simulink model "mainPID"  (R2018b)
settings: Solver=ode5  StartTime=0.0  StopTime=10  RelTol=1e-3
InitFcn:
  | init
values from neighbouring files (symbols this model uses):
  AngDisp = [0 1.57079632679 1.57079632679 1.57079632679 1.57079632679 1.57079632679 0]    [MPCerror.mat]    (also in PIDerror.mat; Q_MPC.m = [0,pi/2,pi/2,pi/2,pi/2,pi/2,0]; Q_PID.m = [0,pi/2,pi/2,pi/2,pi/2,pi/2,0])
  AngVel = [0 0 0 0 0 0 0]    [MPCerror.mat]    (also in PIDerror.mat; Q_MPC.m = [0,0,0,0,0,0,0]; Q_PID.m = [0,0,0,0,0,0,0])
  params = [0.2 3 9.149 36.044 9.149 3 0.2 0.1 0.4 0.4 0.625 0.4 ... (31 elements, 1x31)]    [MPCerror.mat]    (also in PIDerror.mat; Q_MPC.m = [m1,m2,m3,m4,m5,m6,m7,L1,L2,L3,L4,L5,L6,L7,L1c,L2c,L3c,L4c,L; Q_PID.m = [m1,m2,m3,m4,m5,m6,m7,L1,L2,L3,L4,L5,L6,L7,L1c,L2c,L3c,L4c,L)
libraries: simulink x1
settings Model: Creator=Negar Pajooh  LastModifiedBy=Negar Pajooh

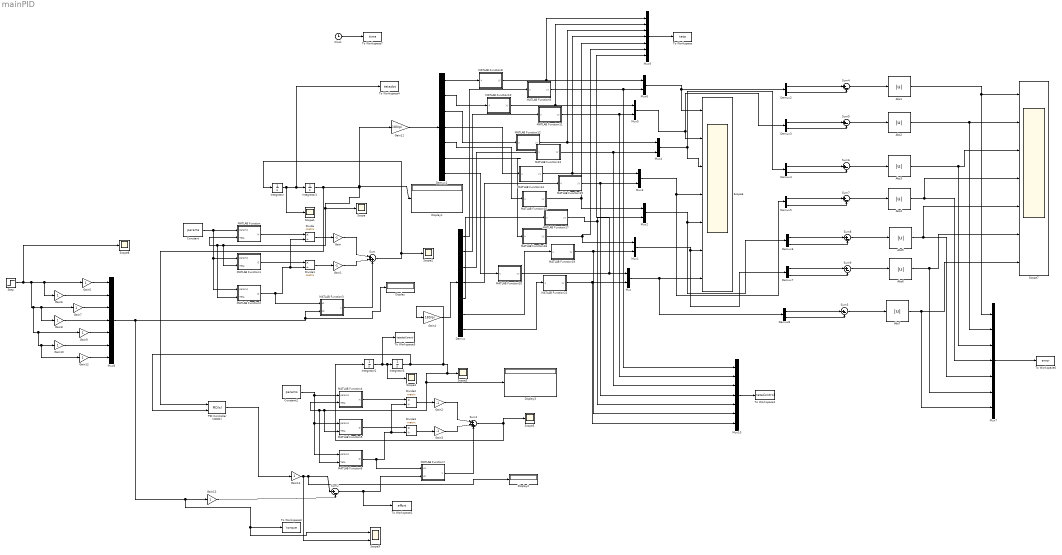
== system mainPID ==
  Abs{1..7} (7 alike) : Abs
  Clock : Clock
  Constant : Constant  Value=params
  Constant2 : Constant  Value=params
  Demux : Demux  Outputs=7
  Demux1 : Demux  Outputs=7
  Demux{2..8} (7 alike) : Demux  Outputs=2
  Display{,1..3} (4 alike) : Display
  Divide{,1..3} (4 alike) : Product  Inputs=*/  Multiplication=Matrix(*)
  Gain{,1..3} (4 alike) : Gain  Gain=-1
  Gain{5..10,12..14} (9 alike) : Gain
  Gain11 : Gain  Gain=180/pi
  Gain4 : Gain  Gain=180/pi
  Integrator : Integrator  InitialCondition=AngVel
  Integrator1 : Integrator  InitialCondition=AngDisp
  Integrator2 : Integrator  InitialCondition=AngVel
  Integrator3 : Integrator  InitialCondition=AngDisp
  MATLAB Function : MATLAB Function  TreatAsAtomicUnit=on
  MATLAB Function1 : MATLAB Function  TreatAsAtomicUnit=on
  MATLAB Function10 : MATLAB Function  TreatAsAtomicUnit=on
  MATLAB Function11 : MATLAB Function  TreatAsAtomicUnit=on
  MATLAB Function12 : MATLAB Function  TreatAsAtomicUnit=on
  MATLAB Function13 : MATLAB Function  TreatAsAtomicUnit=on
  MATLAB Function14 : MATLAB Function  TreatAsAtomicUnit=on
  MATLAB Function15 : MATLAB Function  TreatAsAtomicUnit=on
  MATLAB Function16 : MATLAB Function  TreatAsAtomicUnit=on
  MATLAB Function17 : MATLAB Function  TreatAsAtomicUnit=on
  MATLAB Function18 : MATLAB Function  TreatAsAtomicUnit=on
  MATLAB Function19 : MATLAB Function  TreatAsAtomicUnit=on
  MATLAB Function2 : MATLAB Function  TreatAsAtomicUnit=on
  MATLAB Function20 : MATLAB Function  TreatAsAtomicUnit=on
  MATLAB Function21 : MATLAB Function  TreatAsAtomicUnit=on
  MATLAB Function3 : MATLAB Function  TreatAsAtomicUnit=on
  MATLAB Function4 : MATLAB Function  TreatAsAtomicUnit=on
  MATLAB Function5 : MATLAB Function  TreatAsAtomicUnit=on
  MATLAB Function6 : MATLAB Function  TreatAsAtomicUnit=on
  MATLAB Function7 : MATLAB Function  TreatAsAtomicUnit=on
  MATLAB Function8 : MATLAB Function  TreatAsAtomicUnit=on
  MATLAB Function9 : MATLAB Function  TreatAsAtomicUnit=on
  Mux{,1..6} (7 alike) : Mux  Inputs=2
  Mux{7..10} (4 alike) : Mux  Inputs=7
  PID Controller (2DOF) : simulink/Continuous/PID Controller (2DOF)  Controller=PID  Form=Parallel  TimeDomain=Continuous-time  SampleTime=-1  IntegratorMethod=Forward Euler  FilterMethod=Forward Euler  ControllerParametersSource=internal  P=10  I=0.001  D=0  UseFilter=on  N=100  b=1  c=1  TunerSelectOption=Transfer Function Based (PID Tuner App)  InitialConditionSource=internal  InitialConditionForIntegrator=0  InitialConditionForFilter=0  DifferentiatorICPrevScaledInput=0  ExternalReset=none  TrackingMode=off  Kt=1  LimitOutput=off  UpperSaturationLimit=inf  LowerSaturationLimit=-inf  LinearizeAsGain=on  AntiWindupMode=none  Kb=1  POutMin=[]  POutMax=[]  IOutMin=[]  IOutMax=[]  DOutMin=[]  DOutMax=[]  NOutMin=[]  NOutMax=[]  bOutMin=[]  bOutMax=[]  cOutMin=[]  cOutMax=[]  SumOutMin=[]  SumOutMax=[]  SaturationOutMin=[]  SaturationOutMax=[]  PParamMin=[]  PParamMax=[]  IParamMin=[]  IParamMax=[]  DParamMin=[]  DParamMax=[]  NParamMin=[]  NParamMax=[]  bParamMin=[]  bParamMax=[]  cParamMin=[]  cParamMax=[]  KbParamMin=[]  KbParamMax=[]  KtParamMin=[]  KtParamMax=[]  KbOutMin=[]  KbOutMax=[]  KtOutMin=[]  KtOutMax=[]  IntegratorOutMin=[]  IntegratorOutMax=[]  FilterOutMin=[]  FilterOutMax=[]  SumI1OutMin=[]  SumI1OutMax=[]  SumI2OutMin=[]  SumI2OutMax=[]  SumI3OutMin=[]  SumI3OutMax=[]  SumI4OutMin=[]  SumI4OutMax=[]  SumDOutMin=[]  SumDOutMax=[]  Sum1OutMin=[]  Sum1OutMax=[]  Sum2OutMin=[]  Sum2OutMax=[]  Sum3OutMin=[]  Sum3OutMax=[]  DifferentiatorOutMin=[]  DifferentiatorOutMax=[]  FilterDiffOutCoefMin=[]  FilterDiffOutCoefMax=[]  ReciprocalOutMin=[]  ReciprocalOutMax=[]  SumDenOutMin=[]  SumDenOutMax=[]  SumNumOutMin=[]  SumNumOutMax=[]  DivideOutMin=[]  DivideOutMax=[]  IntegratorContinuousStateAttributes=''  IntegratorStateMustResolveToSignalObject=off  IntegratorRTWStateStorageClass=Auto  FilterContinuousStateAttributes=''  FilterStateMustResolveToSignalObject=off  FilterRTWStateStorageClass=Auto  ParallelPVariant=InternalParameters  IdealPVariant=Disabled  IVariant=InternalParameters  DVariant=InternalParameters  bVariant=InternalParameters  cVariant=InternalParameters  IntegratorVariant=Continuous  SatVariant=Disabled  AWVariant=Passthrough  PCopyVariant=Disabled  TRVariant=Disabled  FdbkBlocksVariant=Forward  IdealPFdbkVariant=Disabled  SatFdbkVariant=Disabled  DerivativeFilterVariant=ContFilter  NVariant=InternalParameters  NCopyVariant=Disabled  FilterICVariant=InternalICsFilter  IntegratorICVariant=InternalICs  ExternalResetVariant=Disabled  TRSumVariant=Passthrough  SumFdbkVariant=Disabled  SumVariant=Sum_PID
  Scope{,1..5,8} (7 alike) : Scope
  Scope6 : Scope  NumInputPorts=7
  Scope7 : Scope  NumInputPorts=7
  Scope9 : Scope  NumInputPorts=2
  Step : Step  SampleTime=0
  Sum : Sum  Inputs=|+++
  Sum1 : Sum  Inputs=|+++
  Sum{2..9} (8 alike) : Sum  Inputs=|+-
  To Workspace : ToWorkspace  VariableName=teta  SampleTime=-1
      settings: Save2DSignal=2-D array (concatenate along first dimension)
  To Workspace1 : ToWorkspace  VariableName=tetaControl  SampleTime=-1
      settings: Save2DSignal=2-D array (concatenate along first dimension)
  To Workspace2 : ToWorkspace  VariableName=effort  SampleTime=-1
      settings: Save2DSignal=2-D array (concatenate along first dimension)
  To Workspace3 : ToWorkspace  VariableName=torque  SampleTime=-1
      settings: Save2DSignal=2-D array (concatenate along first dimension)
  To Workspace4 : ToWorkspace  VariableName=tetadot  SampleTime=-1
      settings: Save2DSignal=2-D array (concatenate along first dimension)
  To Workspace5 : ToWorkspace  VariableName=tetadotControl  SampleTime=-1
      settings: Save2DSignal=2-D array (concatenate along first dimension)
  To Workspace6 : ToWorkspace  VariableName=error  SampleTime=-1
      settings: Save2DSignal=2-D array (concatenate along first dimension)
  To Workspace7 : ToWorkspace  VariableName=time  SampleTime=-1
      settings: Save2DSignal=2-D array (concatenate along first dimension)
  wires:
  Constant/1 -> MATLAB Function2/1(params), MATLAB Function1/1(params), MATLAB Function/1(params)
  Integrator/1 -> Scope1/1, To Workspace4/1, Integrator1/1
  MATLAB Function/1(H) -> Divide/1
  MATLAB Function2/1(D) -> MATLAB Function3/1(u1), Divide/2, Divide1/2
  MATLAB Function1/1(G) -> Divide1/1
  Divide/1 -> Gain/1
  Divide1/1 -> Gain1/1
  Sum/1 -> Integrator/1, Scope2/1
  Gain1/1 -> Sum/2
  Gain/1 -> Sum/1
  Mux8/1 -> Scope9/1, To Workspace3/1, Gain13/1, MATLAB Function3/2(u2), Display/1
  MATLAB Function3/1(y) -> Sum/3
  Divide2/1 -> Gain2/1
  Divide3/1 -> Gain3/1
  MATLAB Function5/1(G) -> Divide3/1
  Gain3/1 -> Sum1/2
  Gain2/1 -> Sum1/1
  Sum1/1 -> Scope5/1, Integrator2/1
  MATLAB Function6/1(D) -> MATLAB Function7/1(u1), Divide2/2, Divide3/2
  Integrator2/1 -> To Workspace5/1, Scope4/1, Integrator3/1
  Constant2/1 -> MATLAB Function6/1(params), MATLAB Function5/1(params), MATLAB Function4/1(params)
  MATLAB Function4/1(H) -> Divide2/1
  MATLAB Function7/1(y) -> Sum1/3
  Sum2/1 -> To Workspace2/1, MATLAB Function7/2(u2)
  Gain11/1 -> Demux1/1
  Gain4/1 -> Demux/1
  Sum4/1 -> Abs1/1
  Demux2/1 -> Sum4/1
  Demux2/2 -> Sum4/2
  Demux3/2 -> Sum5/2
  Demux3/1 -> Sum5/1
  Sum5/1 -> Abs2/1
  Sum6/1 -> Abs3/1
  Demux4/1 -> Sum6/1
  Demux4/2 -> Sum6/2
  Demux5/2 -> Sum7/2
  Demux5/1 -> Sum7/1
  Sum7/1 -> Abs4/1
  Sum8/1 -> Abs5/1
  Demux6/1 -> Sum8/1
  Demux6/2 -> Sum8/2
  Demux7/2 -> Sum9/2
  Demux7/1 -> Sum9/1
  Sum9/1 -> Abs6/1
  Sum3/1 -> Abs7/1
  Demux8/1 -> Sum3/1
  Demux8/2 -> Sum3/2
  Abs2/1 -> Mux7/2, Scope7/2
  Abs3/1 -> Mux7/3, Scope7/3
  Abs4/1 -> Mux7/4, Scope7/4
  Abs6/1 -> Mux7/6, Scope7/6
  Abs7/1 -> Mux7/7, Scope7/7
  Mux7/1 -> To Workspace6/1
  Abs5/1 -> Mux7/5, Scope7/5
  Clock/1 -> To Workspace7/1
  Abs1/1 -> Mux7/1, Scope7/1
  Gain5/1 -> Mux8/1
  Gain6/1 -> Mux8/2
  Gain8/1 -> Mux8/4
  Gain9/1 -> Mux8/5
  Gain10/1 -> Mux8/6
  Gain12/1 -> Mux8/7
  Step/1 -> Scope8/1, Gain12/1, Gain10/1, Gain9/1, Gain8/1, Gain7/1, Gain6/1, Gain5/1
  Gain7/1 -> Mux8/3
  Mux6/1 -> Scope6/1, Demux2/1
  Mux5/1 -> Scope6/2, Demux3/1
  Mux4/1 -> Scope6/3, Demux4/1
  Mux3/1 -> Demux5/1, Scope6/4
  Mux2/1 -> Demux6/1, Scope6/5
  Mux1/1 -> Demux7/1, Scope6/6
  Mux/1 -> Demux8/1, Scope6/7
  Demux1/1 -> MATLAB Function8/1(u)
  Demux/1 -> MATLAB Function9/1(u)
  Demux1/2 -> MATLAB Function10/1(u)
  Demux/2 -> MATLAB Function11/1(u)
  Demux1/3 -> MATLAB Function12/1(u)
  Demux/3 -> MATLAB Function13/1(u)
  Demux1/4 -> MATLAB Function14/1(u)
  Demux/4 -> MATLAB Function15/1(u)
  Demux1/5 -> MATLAB Function16/1(u)
  Demux/5 -> MATLAB Function17/1(u)
  Demux1/6 -> MATLAB Function18/1(u)
  Demux/6 -> MATLAB Function19/1(u)
  Demux1/7 -> MATLAB Function20/1(u)
  Demux/7 -> MATLAB Function21/1(u)
  MATLAB Function8/1(yy) -> Mux9/1, Mux6/1
  MATLAB Function10/1(yy) -> Mux9/2, Mux5/1
  MATLAB Function11/1(yy) -> Mux10/2, Mux5/2
  MATLAB Function12/1(yy) -> Mux9/3, Mux4/1
  MATLAB Function14/1(yy) -> Mux3/1, Mux9/4
  MATLAB Function16/1(yy) -> Mux2/1, Mux9/5
  MATLAB Function17/1(yy) -> Mux2/2, Mux10/5
  MATLAB Function18/1(yy) -> Mux1/1, Mux9/6
  MATLAB Function19/1(yy) -> Mux10/6, Mux1/2
  MATLAB Function20/1(yy) -> Mux9/7, Mux/1
  MATLAB Function21/1(yy) -> Mux10/7, Mux/2
  Mux9/1 -> To Workspace/1
  Mux10/1 -> To Workspace1/1
  MATLAB Function9/1(yy) -> Mux10/1, Mux6/2
  MATLAB Function13/1(yy) -> Mux10/3, Mux4/2
  MATLAB Function15/1(yy) -> Mux10/4, Mux3/2
  Gain13/1 -> Sum2/2
  Gain14/1 -> Scope9/2, Sum2/1, Display2/1
  Integrator3/1 -> PID Controller (2DOF)/2, MATLAB Function5/2(Teta), MATLAB Function6/2(Teta), MATLAB Function4/2(Teta), Display3/1, Scope3/1, Gain4/1
  Integrator1/1 -> PID Controller (2DOF)/1, Scope/1, MATLAB Function1/2(Teta), MATLAB Function2/2(Teta), MATLAB Function/2(Teta), Gain11/1, Display1/1
  PID Controller (2DOF)/1 -> Gain14/1

== matlab function mainPID/MATLAB Function1 ==
  data: params input; G output; Teta input
function G=G(params,Teta)
%% params
m1=params(1);m2=params(2);m3=params(3);m4=params(4);m5=params(5);m6=params(6);m7=params(7);
L1=params(8);L2=params(9);L3=params(10);L4=params(11);L5=params(12);L6=params(13);L7=params(14);
L1c=params(22);L2c=params(23);L3c=params(24);L4c=params(25);L5c=params(26);L6c=params(27);L7c=params(28);
I1=params(15);I2=params(16);I3=params(17);I4=params(18);I5=params(19);I6=params(20);I7=params(21);
h=params(29);k=params(30);g=params(31);
%% Teta
teta1=Teta(1);
teta2=Teta(2);
teta3=Teta(3);
teta4=Teta(4);
teta5=Teta(5);
teta6=Teta(6);
teta7=Teta(7);
%%
G1=g*cos(teta1)*(m1*L1c+m2*L1+m3*L1+m4*L1+m5*L1+m6*L1+m7*L1)-...
    g*sin(teta1)*(m2*h+m3*h+m4*h+m5*h+m6*h+m7*h);
G2=g*cos(teta2)*(m2*L2c+m3*L2+m4*L2+m6*L2+m7*L2);
G3=g*cos(teta3)*(m3*L3c+m4*L3+m5*L3+m6*L3+m7*L3);
G4=g*cos(teta4)*(m4*L4c);
G5=-g*cos(teta5)*(m5*L5-m5*L5c+m6*L5+m7*L5);
G6=-g*cos(teta6)*(m6*L6-m6*L6c+m7*L6);
G7=g*cos(teta7)*(m7*L7c)+g*sin(teta7)*(m7*k);
%%
G=[G1;G2;G3;G4;G5;G6;G7]';
% G=G';
end

== matlab function mainPID/MATLAB Function ==
  data: params input; H output; Teta input
function H=H(params,Teta)
%% params
m1=params(1);m2=params(2);m3=params(3);m4=params(4);m5=params(5);m6=params(6);m7=params(7);
L1=params(8);L2=params(9);L3=params(10);L4=params(11);L5=params(12);L6=params(13);L7=params(14);
L1c=params(22);L2c=params(23);L3c=params(24);L4c=params(25);L5c=params(26);L6c=params(27);L7c=params(28);
I1=params(15);I2=params(16);I3=params(17);I4=params(18);I5=params(19);I6=params(20);I7=params(21);
h=params(29);k=params(30);g=params(31);
%% Teta
teta1=Teta(1);
teta2=Teta(2);
teta3=Teta(3);
teta4=Teta(4);
teta5=Teta(5);
teta6=Teta(6);
teta7=Teta(7);
HH=zeros(7);
%%
HH(1,1)=0;
HH(1,2)=(-m2*h*L2c-m3*h*L2-m4*h*L2-m5*h*L2-m6*h*L2-m7*h*L2)*cos(teta1+teta2)+...
-(m2*L1*L2c+m3*L1*L2+m4*L1*L2+m5*L1*L2+m6*L1*L2+m7*L1*L2)*sin(teta1+teta2);
HH(1,3)=(-m3*h*L3c-m4*h*L3-m5*h*L3-m6*h*L3-m7*h*L3)*cos(teta1+teta3)-...
(m3*L1*L3c+m4*L1*L3+m5*L1*L3+m6*L1*L3+m7*L1*L3)*sin(teta1+teta3);
HH(1,4)=(-m4*h*L4c)*cos(teta1+teta4)-(m4*L1*L4c)*sin(teta1+teta4);
HH(1,5)=-(m5*h*L5-m5*h*L5c+m6*h*L5+m7*h*L5)*cos(teta1-teta5)+...
(-m5*L1*L5+m5*L1*L5c-m6*L1*L5-m7*L1*L5)*sin(teta1-teta5);
HH(1,6)=-(m6*h*L6-m6*h*L6c+m7*h*L6)*cos(teta1-teta6)+...
(-m6*L1*L6+m6*L1*L6c-m7*L1*L6c)*sin(teta1-teta6);
HH(1,7)=(m7*L1*k-m7*h*L7c)*cos(teta1+teta7)-...
(m7*L1*L7c+m7*h*k)*sin(teta1+teta7);
%%
HH(2,1)=HH(1,2);
HH(2,2)=0;
HH(2,3)=(m3*L2*L3c+m4*L2*L3+m5*L2*L3+m6*L2*L3+m7*L2*L3)*sin(teta2-teta3);
HH(2,4)=m4*L2*L4c*sin(teta2-teta4);
HH(2,5)=-(-m5*L2*L5+m5*L2*L5c-m6*L2*L5-m7*L2*L5)*sin(teta2+teta5);
HH(2,6)=-(-m6*L2*L6+m6*L2*L6c-m7*L2*L6)*sin(teta2+teta6);
HH(2,7)=-(-m7*L2*k)*cos(teta2-teta7)+m7*L2*L7c*sin(teta2-teta7);
%%
HH(3,1)=HH(1,3);
HH(3,2)=-HH(2,3);
HH(3,3)=0;
HH(3,4)=m4*L3*L4c*sin(teta3-teta4);
HH(3,5)=-(-m5*L3*L5+m5*L3*L5c-m7*L3*L6)*sin(teta3+teta5);
HH(3,6)=-(-m6*L3*L6+m6*L3*L6c-m7*L3*L6)*sin(teta3+teta6);
HH(3,7)=-(-m7*L3*k)*cos(teta3-teta7)+m7*L3*L7c*sin(teta3-teta7);
%%
HH(4,1)=HH(1,4);
HH(4,2)=-HH(2,4);
HH(4,3)=-HH(3,4);
HH(4,4)=0;
HH(4,5)=0;
HH(4,6)=0;
HH(4,7)=0;
%%
HH(5,1)=HH(1,5);
HH(5,2)=HH(2,5);
HH(5,3)=HH(3,5);
HH(5,4)=0;
HH(5,5)=0;
HH(5,6)=(m6*L5*L6-m6*L5*L6c+m7*L5*L6)*sin(teta5-teta6);
HH(5,7)=-m7*L5*k*cos(teta5+teta7)+m7*L5*L7c*sin(teta5+teta7);
%%
HH(6,1)=-HH(1,6);
HH(6,2)=HH(2,6);
HH(6,3)=HH(3,6);
HH(6,4)=0;
HH(6,5)=-HH(5,6);
HH(6,6)=0;
HH(6,7)=-m7*L5*k*cos(teta6+teta7)+m7*L5*L7c*sin(teta5+teta7);
%%
HH(7,1)=HH(1,7);
HH(7,2)=-HH(2,7);
HH(7,3)=-HH(3,7);
HH(7,4)=0;
HH(7,5)=HH(5,7);
HH(7,6)=HH(6,7);
HH(7,7)=0;
%%
H=zeros(1,7);
for i=1:7
H(1,i)=HH(i,1)+HH(i,2)+HH(i,3)+HH(i,4)+HH(i,5)+HH(i,6)+HH(i,7);
end
% H=H';
%%
end

== matlab function mainPID/MATLAB Function2 ==
  data: params input; D output; Teta input
function D=D(params,Teta)
%% params
% m1=params.m1;m2=params.m2;m3=params.m3;m4=params.m4;m5=params.m5;m6=params.m6;m7=params.m7;
% L1=params.L1;L2=params.L2;L3=params.L3;L4=params.L4;L5=params.L5;L6=params.L6;L7=params.L7;
% L1c=params.L1c;L2c=params.L2c;L3c=params.L3c;L4c=params.L4c;L5c=params.L5c;L6c=params.L6c;L7c=params.L7c;
% I1=params.I1;I2=params.I2;I3=params.I3;I4=params.I4;I5=params.I5;I6=params.I6;I7=params.I7;
% h=params.h;
% k=params.k;
% g=params.g;
m1=params(1);m2=params(2);m3=params(3);m4=params(4);m5=params(5);m6=params(6);m7=params(7);
L1=params(8);L2=params(9);L3=params(10);L4=params(11);L5=params(12);L6=params(13);L7=params(14);
L1c=params(22);L2c=params(23);L3c=params(24);L4c=params(25);L5c=params(26);L6c=params(27);L7c=params(28);
I1=params(15);I2=params(16);I3=params(17);I4=params(18);I5=params(19);I6=params(20);I7=params(21);
h=params(29);
k=params(30);
g=params(31);
%% Teta
teta1=Teta(1);
teta2=Teta(2);
teta3=Teta(3);
teta4=Teta(4);
teta5=Teta(5);
teta6=Teta(6);
teta7=Teta(7);
D=zeros(7);
%%
D(1,1)=m1*(L1c^2)+I1+m2*(L1^2)+m2*(h^2)+m3*(L1^2)+m3*(h^2)+m4*(L1^2)+...
    m4*(h^2)+m5*(L1^2)+m5*(h^2)+m6*(L1^2)+m6*(h^2)+m7*(L1^2)+m7*(h^2);
%
D121=m2*L1*L2c+m3*L1*L2+m4*L2*L1+m5*L1*L2+m6*L1*L2+m7*L1*L2;
D122=-m2*h*L2c-m3*h*L2-m4*h*L2-m5*h*L2-m6*h*L2-m7*h*L2;
D(1,2)=D121*cos(teta1+teta2)+D122*sin(teta1+teta2);
%
D131=m3*L1*L3c+m4*L1*L3+m5*L1*L3+m6*L1*L3+m7*L1*L3;
D132=-m3*h*L3c-m4*h*L3-m5*h*L3-m6*h*L3-m7*h*L3;
D(1,3)=D131*cos(teta1+teta3)+D132*sin(teta1+teta3);
%
D(1,4)=m4*L1*L4c*cos(teta1+teta4)-m4*h*L4c*sin(teta1+teta4);
%
D151=-m5*L1*L5+m5*L1*L5c-m6*L1*L5-m7*L1*L5;
D152=m5*h*L5-m5*h*L5c+m6*h*L5+m7*h*L5;
D(1,5)=D151*cos(teta1-teta5)+D152*sin(teta1-teta5);
%
D161=-m6*L1*L6+m6*L1*L6c-m7*L1*L6;
D162=m6*L6*h-m6*h*L6c+m7*h*L6;
D(1,6)=D161*cos(teta1-teta6)+D162*sin(teta1-teta6);
%
D(1,7)=(m7*L1*k-m7*h*L7c)*sin(teta1+teta7)+...
    (m7*L1*L7c+m7*h*k)*cos(teta1+teta7);
%%
D(2,1)=D(1,2);
D(2,2)=m2*(L2c^2)+I2+m3*(L2^2)+m5*(L2^2)+m6*(L2^2)+m7*(L2^2);
D(2,3)=(m3*L2*L3c+m4*L2*L3+m5*L2*L3+m6*L2*L3+m7*L2*L3)*cos(teta2-teta3);
D(2,4)=m4*L2*L4c*cos(teta2-teta4);
D(2,5)=(-m5*L2*L5+m5*L2*L5c-m6*L2*L5-m7*L2*L5)*cos(teta2+teta5);
D(2,6)=(-m6*L2*L6+m6*L2*L6c-m7*L2*L6)*cos(teta2+teta6);
D(2,7)=-m7*L2*k*sin(teta2-teta7)+m7*L2*L7c*cos(teta2-teta7);
%%
D(3,1)=D(1,3);
D(3,2)=D(2,3);
D(3,3)=m3*(L3c^2)+I3+m4*(L3^2)+m5*(L3^2)+m6*(L3^2)+m7*(L3^2);
D(3,4)=m4*L3*L4c*cos(teta3-teta4);
D(3,5)=(-m5*L3*L5+m5*L3*L5c-m6*L3*L5-m7*L3*L5)*cos(teta3+teta5);
D(3,6)=(-m6*L3*L6+m6*L3*L6c-m7*L3*L6)*cos(teta3+teta6);
D(3,7)=-m7*L3*k*sin(teta3-teta7)+m7*L3*L7c*cos(teta3-teta7);
%%
D(4,1)=D(1,4);
D(4,2)=D(2,4);
D(4,3)=D(3,4);
D(4,4)=m4*(L4c^2)+I4;
D(4,5)=0;
D(4,6)=0;
D(4,7)=0;
%%
D(5,1)=D(1,5);
D(5,2)=D(2,5);
D(5,3)=D(3,5);
D(5,4)=D(4,5);
D(5,5)=m5*(L5^2)+m5*(L5c^2)-2*m5*L5*L5c+I5+m6*(L5^2)+m7*(L5^2);
D(5,6)=(m6*L5*L6-m6*L6*L6c+m7*L5*L6)*cos(teta5-teta6);
D(5,7)=-m7*L5*k*sin(teta5+teta7)-m7*L5*L7c*cos(teta5+teta7);
%%
D(6,1)=D(1,6);
D(6,2)=D(2,6);
D(6,3)=D(3,6);
D(6,4)=D(4,6);
D(6,5)=D(5,6);
D(6,6)=m6*(L6^2)+m2*(L5c^2)-2*m5*L5*L5c+I5+m6*(L5^2)+m7*(L5^2);
D(6,7)=-m7*L5*k*sin(teta5+teta7)-m7*L5*L7c*cos(teta5+teta7);
%%
D(7,1)=D(1,7);
D(7,2)=D(2,7);
D(7,3)=D(3,7);
D(7,4)=D(4,7);
D(7,5)=D(5,7);
D(7,6)=D(6,7);
D(7,7)=m7*(k^2)+m7*(L7c^2)+I7;
%%


end

== matlab function mainPID/MATLAB Function3 ==
  data: u1 input; y output; u2 input
function y = fcn(u1,u2)

y = inv(u1)*u2;

== matlab function mainPID/MATLAB Function4 ==
  data: params input; H output; Teta input
function H=H(params,Teta)
%% params
m1=params(1);m2=params(2);m3=params(3);m4=params(4);m5=params(5);m6=params(6);m7=params(7);
L1=params(8);L2=params(9);L3=params(10);L4=params(11);L5=params(12);L6=params(13);L7=params(14);
L1c=params(22);L2c=params(23);L3c=params(24);L4c=params(25);L5c=params(26);L6c=params(27);L7c=params(28);
I1=params(15);I2=params(16);I3=params(17);I4=params(18);I5=params(19);I6=params(20);I7=params(21);
h=params(29);k=params(30);g=params(31);
%% Teta
teta1=Teta(1);
teta2=Teta(2);
teta3=Teta(3);
teta4=Teta(4);
teta5=Teta(5);
teta6=Teta(6);
teta7=Teta(7);
HH=zeros(7);
%%
HH(1,1)=0;
HH(1,2)=(-m2*h*L2c-m3*h*L2-m4*h*L2-m5*h*L2-m6*h*L2-m7*h*L2)*cos(teta1+teta2)+...
-(m2*L1*L2c+m3*L1*L2+m4*L1*L2+m5*L1*L2+m6*L1*L2+m7*L1*L2)*sin(teta1+teta2);
HH(1,3)=(-m3*h*L3c-m4*h*L3-m5*h*L3-m6*h*L3-m7*h*L3)*cos(teta1+teta3)-...
(m3*L1*L3c+m4*L1*L3+m5*L1*L3+m6*L1*L3+m7*L1*L3)*sin(teta1+teta3);
HH(1,4)=(-m4*h*L4c)*cos(teta1+teta4)-(m4*L1*L4c)*sin(teta1+teta4);
HH(1,5)=-(m5*h*L5-m5*h*L5c+m6*h*L5+m7*h*L5)*cos(teta1-teta5)+...
(-m5*L1*L5+m5*L1*L5c-m6*L1*L5-m7*L1*L5)*sin(teta1-teta5);
HH(1,6)=-(m6*h*L6-m6*h*L6c+m7*h*L6)*cos(teta1-teta6)+...
(-m6*L1*L6+m6*L1*L6c-m7*L1*L6c)*sin(teta1-teta6);
HH(1,7)=(m7*L1*k-m7*h*L7c)*cos(teta1+teta7)-...
(m7*L1*L7c+m7*h*k)*sin(teta1+teta7);
%%
HH(2,1)=HH(1,2);
HH(2,2)=0;
HH(2,3)=(m3*L2*L3c+m4*L2*L3+m5*L2*L3+m6*L2*L3+m7*L2*L3)*sin(teta2-teta3);
HH(2,4)=m4*L2*L4c*sin(teta2-teta4);
HH(2,5)=-(-m5*L2*L5+m5*L2*L5c-m6*L2*L5-m7*L2*L5)*sin(teta2+teta5);
HH(2,6)=-(-m6*L2*L6+m6*L2*L6c-m7*L2*L6)*sin(teta2+teta6);
HH(2,7)=-(-m7*L2*k)*cos(teta2-teta7)+m7*L2*L7c*sin(teta2-teta7);
%%
HH(3,1)=HH(1,3);
HH(3,2)=-HH(2,3);
HH(3,3)=0;
HH(3,4)=m4*L3*L4c*sin(teta3-teta4);
HH(3,5)=-(-m5*L3*L5+m5*L3*L5c-m7*L3*L6)*sin(teta3+teta5);
HH(3,6)=-(-m6*L3*L6+m6*L3*L6c-m7*L3*L6)*sin(teta3+teta6);
HH(3,7)=-(-m7*L3*k)*cos(teta3-teta7)+m7*L3*L7c*sin(teta3-teta7);
%%
HH(4,1)=HH(1,4);
HH(4,2)=-HH(2,4);
HH(4,3)=-HH(3,4);
HH(4,4)=0;
HH(4,5)=0;
HH(4,6)=0;
HH(4,7)=0;
%%
HH(5,1)=HH(1,5);
HH(5,2)=HH(2,5);
HH(5,3)=HH(3,5);
HH(5,4)=0;
HH(5,5)=0;
HH(5,6)=(m6*L5*L6-m6*L5*L6c+m7*L5*L6)*sin(teta5-teta6);
HH(5,7)=-m7*L5*k*cos(teta5+teta7)+m7*L5*L7c*sin(teta5+teta7);
%%
HH(6,1)=-HH(1,6);
HH(6,2)=HH(2,6);
HH(6,3)=HH(3,6);
HH(6,4)=0;
HH(6,5)=-HH(5,6);
HH(6,6)=0;
HH(6,7)=-m7*L5*k*cos(teta6+teta7)+m7*L5*L7c*sin(teta5+teta7);
%%
HH(7,1)=HH(1,7);
HH(7,2)=-HH(2,7);
HH(7,3)=-HH(3,7);
HH(7,4)=0;
HH(7,5)=HH(5,7);
HH(7,6)=HH(6,7);
HH(7,7)=0;
%%
H=zeros(1,7);
for i=1:7
H(1,i)=HH(i,1)+HH(i,2)+HH(i,3)+HH(i,4)+HH(i,5)+HH(i,6)+HH(i,7);
end
% H=H';
%%
end

== matlab function mainPID/MATLAB Function5 ==
  data: params input; G output; Teta input
function G=G(params,Teta)
%% params
m1=params(1);m2=params(2);m3=params(3);m4=params(4);m5=params(5);m6=params(6);m7=params(7);
L1=params(8);L2=params(9);L3=params(10);L4=params(11);L5=params(12);L6=params(13);L7=params(14);
L1c=params(22);L2c=params(23);L3c=params(24);L4c=params(25);L5c=params(26);L6c=params(27);L7c=params(28);
I1=params(15);I2=params(16);I3=params(17);I4=params(18);I5=params(19);I6=params(20);I7=params(21);
h=params(29);k=params(30);g=params(31);
%% Teta
teta1=Teta(1);
teta2=Teta(2);
teta3=Teta(3);
teta4=Teta(4);
teta5=Teta(5);
teta6=Teta(6);
teta7=Teta(7);
%%
G1=g*cos(teta1)*(m1*L1c+m2*L1+m3*L1+m4*L1+m5*L1+m6*L1+m7*L1)-...
    g*sin(teta1)*(m2*h+m3*h+m4*h+m5*h+m6*h+m7*h);
G2=g*cos(teta2)*(m2*L2c+m3*L2+m4*L2+m6*L2+m7*L2);
G3=g*cos(teta3)*(m3*L3c+m4*L3+m5*L3+m6*L3+m7*L3);
G4=g*cos(teta4)*(m4*L4c);
G5=-g*cos(teta5)*(m5*L5-m5*L5c+m6*L5+m7*L5);
G6=-g*cos(teta6)*(m6*L6-m6*L6c+m7*L6);
G7=g*cos(teta7)*(m7*L7c)+g*sin(teta7)*(m7*k);
%%
G=[G1;G2;G3;G4;G5;G6;G7]';
% G=G';
end

== matlab function mainPID/MATLAB Function6 ==
  data: params input; D output; Teta input
function D=D(params,Teta)
%% params
% m1=params.m1;m2=params.m2;m3=params.m3;m4=params.m4;m5=params.m5;m6=params.m6;m7=params.m7;
% L1=params.L1;L2=params.L2;L3=params.L3;L4=params.L4;L5=params.L5;L6=params.L6;L7=params.L7;
% L1c=params.L1c;L2c=params.L2c;L3c=params.L3c;L4c=params.L4c;L5c=params.L5c;L6c=params.L6c;L7c=params.L7c;
% I1=params.I1;I2=params.I2;I3=params.I3;I4=params.I4;I5=params.I5;I6=params.I6;I7=params.I7;
% h=params.h;
% k=params.k;
% g=params.g;
m1=params(1);m2=params(2);m3=params(3);m4=params(4);m5=params(5);m6=params(6);m7=params(7);
L1=params(8);L2=params(9);L3=params(10);L4=params(11);L5=params(12);L6=params(13);L7=params(14);
L1c=params(22);L2c=params(23);L3c=params(24);L4c=params(25);L5c=params(26);L6c=params(27);L7c=params(28);
I1=params(15);I2=params(16);I3=params(17);I4=params(18);I5=params(19);I6=params(20);I7=params(21);
h=params(29);
k=params(30);
g=params(31);
%% Teta
teta1=Teta(1);
teta2=Teta(2);
teta3=Teta(3);
teta4=Teta(4);
teta5=Teta(5);
teta6=Teta(6);
teta7=Teta(7);
D=zeros(7);
%%
D(1,1)=m1*(L1c^2)+I1+m2*(L1^2)+m2*(h^2)+m3*(L1^2)+m3*(h^2)+m4*(L1^2)+...
    m4*(h^2)+m5*(L1^2)+m5*(h^2)+m6*(L1^2)+m6*(h^2)+m7*(L1^2)+m7*(h^2);
%
D121=m2*L1*L2c+m3*L1*L2+m4*L2*L1+m5*L1*L2+m6*L1*L2+m7*L1*L2;
D122=-m2*h*L2c-m3*h*L2-m4*h*L2-m5*h*L2-m6*h*L2-m7*h*L2;
D(1,2)=D121*cos(teta1+teta2)+D122*sin(teta1+teta2);
%
D131=m3*L1*L3c+m4*L1*L3+m5*L1*L3+m6*L1*L3+m7*L1*L3;
D132=-m3*h*L3c-m4*h*L3-m5*h*L3-m6*h*L3-m7*h*L3;
D(1,3)=D131*cos(teta1+teta3)+D132*sin(teta1+teta3);
%
D(1,4)=m4*L1*L4c*cos(teta1+teta4)-m4*h*L4c*sin(teta1+teta4);
%
D151=-m5*L1*L5+m5*L1*L5c-m6*L1*L5-m7*L1*L5;
D152=m5*h*L5-m5*h*L5c+m6*h*L5+m7*h*L5;
D(1,5)=D151*cos(teta1-teta5)+D152*sin(teta1-teta5);
%
D161=-m6*L1*L6+m6*L1*L6c-m7*L1*L6;
D162=m6*L6*h-m6*h*L6c+m7*h*L6;
D(1,6)=D161*cos(teta1-teta6)+D162*sin(teta1-teta6);
%
D(1,7)=(m7*L1*k-m7*h*L7c)*sin(teta1+teta7)+...
    (m7*L1*L7c+m7*h*k)*cos(teta1+teta7);
%%
D(2,1)=D(1,2);
D(2,2)=m2*(L2c^2)+I2+m3*(L2^2)+m5*(L2^2)+m6*(L2^2)+m7*(L2^2);
D(2,3)=(m3*L2*L3c+m4*L2*L3+m5*L2*L3+m6*L2*L3+m7*L2*L3)*cos(teta2-teta3);
D(2,4)=m4*L2*L4c*cos(teta2-teta4);
D(2,5)=(-m5*L2*L5+m5*L2*L5c-m6*L2*L5-m7*L2*L5)*cos(teta2+teta5);
D(2,6)=(-m6*L2*L6+m6*L2*L6c-m7*L2*L6)*cos(teta2+teta6);
D(2,7)=-m7*L2*k*sin(teta2-teta7)+m7*L2*L7c*cos(teta2-teta7);
%%
D(3,1)=D(1,3);
D(3,2)=D(2,3);
D(3,3)=m3*(L3c^2)+I3+m4*(L3^2)+m5*(L3^2)+m6*(L3^2)+m7*(L3^2);
D(3,4)=m4*L3*L4c*cos(teta3-teta4);
D(3,5)=(-m5*L3*L5+m5*L3*L5c-m6*L3*L5-m7*L3*L5)*cos(teta3+teta5);
D(3,6)=(-m6*L3*L6+m6*L3*L6c-m7*L3*L6)*cos(teta3+teta6);
D(3,7)=-m7*L3*k*sin(teta3-teta7)+m7*L3*L7c*cos(teta3-teta7);
%%
D(4,1)=D(1,4);
D(4,2)=D(2,4);
D(4,3)=D(3,4);
D(4,4)=m4*(L4c^2)+I4;
D(4,5)=0;
D(4,6)=0;
D(4,7)=0;
%%
D(5,1)=D(1,5);
D(5,2)=D(2,5);
D(5,3)=D(3,5);
D(5,4)=D(4,5);
D(5,5)=m5*(L5^2)+m5*(L5c^2)-2*m5*L5*L5c+I5+m6*(L5^2)+m7*(L5^2);
D(5,6)=(m6*L5*L6-m6*L6*L6c+m7*L5*L6)*cos(teta5-teta6);
D(5,7)=-m7*L5*k*sin(teta5+teta7)-m7*L5*L7c*cos(teta5+teta7);
%%
D(6,1)=D(1,6);
D(6,2)=D(2,6);
D(6,3)=D(3,6);
D(6,4)=D(4,6);
D(6,5)=D(5,6);
D(6,6)=m6*(L6^2)+m2*(L5c^2)-2*m5*L5*L5c+I5+m6*(L5^2)+m7*(L5^2);
D(6,7)=-m7*L5*k*sin(teta5+teta7)-m7*L5*L7c*cos(teta5+teta7);
%%
D(7,1)=D(1,7);
D(7,2)=D(2,7);
D(7,3)=D(3,7);
D(7,4)=D(4,7);
D(7,5)=D(5,7);
D(7,6)=D(6,7);
D(7,7)=m7*(k^2)+m7*(L7c^2)+I7;
%%


end

== matlab function mainPID/MATLAB Function7 ==
  data: u1 input; y output; u2 input
function y = fcn(u1,u2)

y = inv(u1)*u2;

== matlab function mainPID/MATLAB Function8 ==
  data: u input; yy output
function yy = fcn(u)
m=mod(u,360);
y=0;
% if 45<m && m<=90
%   y=90-m;
if 90<m && m<=180
    y=180-m;
    elseif 180<m && m<=270
        y=270-m;
        elseif 270<m && m<=360
           y=360-m;
elseif m<=90
    y=m;
end
yy=y;
end

== matlab function mainPID/MATLAB Function9 ==
  data: u input; yy output
function yy = fcn(u)
m=mod(u,360);
y=0;
% if 45<m && m<=90
%   y=90-m;
if 90<m && m<=180
    y=180-m;
    elseif 180<m && m<=270
        y=270-m;
        elseif 270<m && m<=360
           y=360-m;
elseif m<=90
    y=m;
end
yy=y;
end

== matlab function mainPID/MATLAB Function10 ==
  data: u input; yy output
function yy = fcn(u)
m=mod(u,360);
y=0;
% if 45<m && m<=90
%   y=90-m;
if 90<m && m<=180
    y=180-m;
    elseif 180<m && m<=270
        y=270-m;
        elseif 270<m && m<=360
           y=360-m;
elseif m<=90
    y=m;
end
yy=y;
end

== matlab function mainPID/MATLAB Function11 ==
  data: u input; yy output
function yy = fcn(u)
m=mod(u,360);
y=0;
% if 45<m && m<=90
%   y=90-m;
if 90<m && m<=180
    y=180-m;
    elseif 180<m && m<=270
        y=270-m;
        elseif 270<m && m<=360
           y=360-m;
elseif m<=90
    y=m;
end
yy=y;
end

== matlab function mainPID/MATLAB Function12 ==
  data: u input; yy output
function yy = fcn(u)
m=mod(u,360);
y=0;
% if 45<m && m<=90
%   y=90-m;
if 90<m && m<=180
    y=180-m;
    elseif 180<m && m<=270
        y=270-m;
        elseif 270<m && m<=360
           y=360-m;
elseif m<=90
    y=m;
end
yy=y;
end

== matlab function mainPID/MATLAB Function13 ==
  data: u input; yy output
function yy = fcn(u)
m=mod(u,360);
y=0;
% if 45<m && m<=90
%   y=90-m;
if 90<m && m<=180
    y=180-m;
    elseif 180<m && m<=270
        y=270-m;
        elseif 270<m && m<=360
           y=360-m;
elseif m<=90
    y=m;
end
yy=y;
end

== matlab function mainPID/MATLAB Function14 ==
  data: u input; yy output
function yy = fcn(u)
m=mod(u,360);
y=0;
% if 45<m && m<=90
%   y=90-m;
if 90<m && m<=180
    y=180-m;
    elseif 180<m && m<=270
        y=270-m;
        elseif 270<m && m<=360
           y=360-m;
elseif m<=90
    y=m;
end
yy=y;
end

== matlab function mainPID/MATLAB Function15 ==
  data: u input; yy output
function yy = fcn(u)
m=mod(u,360);
y=0;
% if 45<m && m<=90
%   y=90-m;
if 90<m && m<=180
    y=180-m;
    elseif 180<m && m<=270
        y=270-m;
        elseif 270<m && m<=360
           y=360-m;
elseif m<=90
    y=m;
end
yy=y;
end

== matlab function mainPID/MATLAB Function16 ==
  data: u input; yy output
function yy = fcn(u)
m=mod(u,360);
y=0;
% if 45<m && m<=90
%   y=90-m;
if 90<m && m<=180
    y=180-m;
    elseif 180<m && m<=270
        y=270-m;
        elseif 270<m && m<=360
           y=360-m;
elseif m<=90
    y=m;
end
yy=y;
end

== matlab function mainPID/MATLAB Function17 ==
  data: u input; yy output
function yy = fcn(u)
m=mod(u,360);
y=0;
% if 45<m && m<=90
%   y=90-m;
if 90<m && m<=180
    y=180-m;
    elseif 180<m && m<=270
        y=270-m;
        elseif 270<m && m<=360
           y=360-m;
elseif m<=90
    y=m;
end
yy=y;
end

== matlab function mainPID/MATLAB Function18 ==
  data: u input; yy output
function yy = fcn(u)
m=mod(u,360);
y=0;
% if 45<m && m<=90
%   y=90-m;
if 90<m && m<=180
    y=180-m;
    elseif 180<m && m<=270
        y=270-m;
        elseif 270<m && m<=360
           y=360-m;
elseif m<=90
    y=m;
end
yy=y;
end

== matlab function mainPID/MATLAB Function19 ==
  data: u input; yy output
function yy = fcn(u)
m=mod(u,360);
y=0;
% if 45<m && m<=90
%   y=90-m;
if 90<m && m<=180
    y=180-m;
    elseif 180<m && m<=270
        y=270-m;
        elseif 270<m && m<=360
           y=360-m;
elseif m<=90
    y=m;
end
yy=y;
end

== matlab function mainPID/MATLAB Function20 ==
  data: u input; yy output
function yy = fcn(u)
m=mod(u,360);
y=0;
% if 45<m && m<=90
%   y=90-m;
if 90<m && m<=180
    y=180-m;
    elseif 180<m && m<=270
        y=270-m;
        elseif 270<m && m<=360
           y=360-m;
elseif m<=90
    y=m;
end
yy=y;
end

== matlab function mainPID/MATLAB Function21 ==
  data: u input; yy output
function yy = fcn(u)
m=mod(u,360);
y=0;
% if 45<m && m<=90
%   y=90-m;
if 90<m && m<=180
    y=180-m;
    elseif 180<m && m<=270
        y=270-m;
        elseif 270<m && m<=360
           y=360-m;
elseif m<=90
    y=m;
end
yy=y;
end
